simulink model "VF_Speed"  (R2023b)
settings: Solver=ode23  StartTime=0.0  StopTime=4  MaxStep=1e-6  RelTol=1e-4
InitFcn:
  | Pn = 4;
  | Ld = 5.25e-3;
  | Lq = 12e-3;
  | R = 0.958;
  | flux = 0.1827;
  | J = 0.003;
  | B = 0.008;
  | Vdc = 311;
  | fpwm = 10e3;
  | Ts = 1e-5;
model workspace: external: MATLAB File D:\Simulink\Study\PMSM建模第三章\VF_Params.m (data not in the file)
libraries: spsDCVoltageSourceLib x1, powerlib_extras x1, spsPermanentMagnetSynchronousMachineLib x1, simulink x1, spsUniversalBridgeLib x1, spspowerguiLib x1
settings Model: Creator=123  LastModifiedBy=123
settings ModelReferenceCC: EnableRefExpFcnMdlSchedulingChecks=on

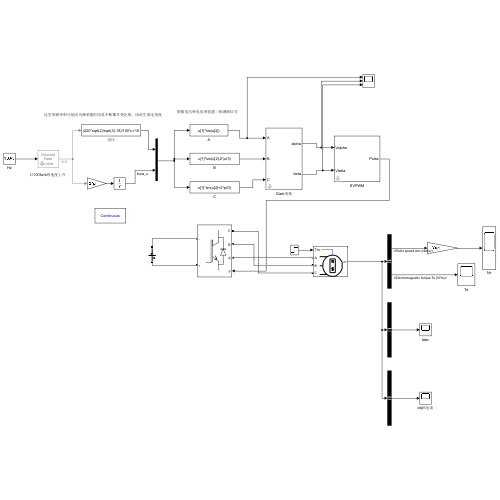
[thumbnail: Simulink's stored preview of the top-level diagram]
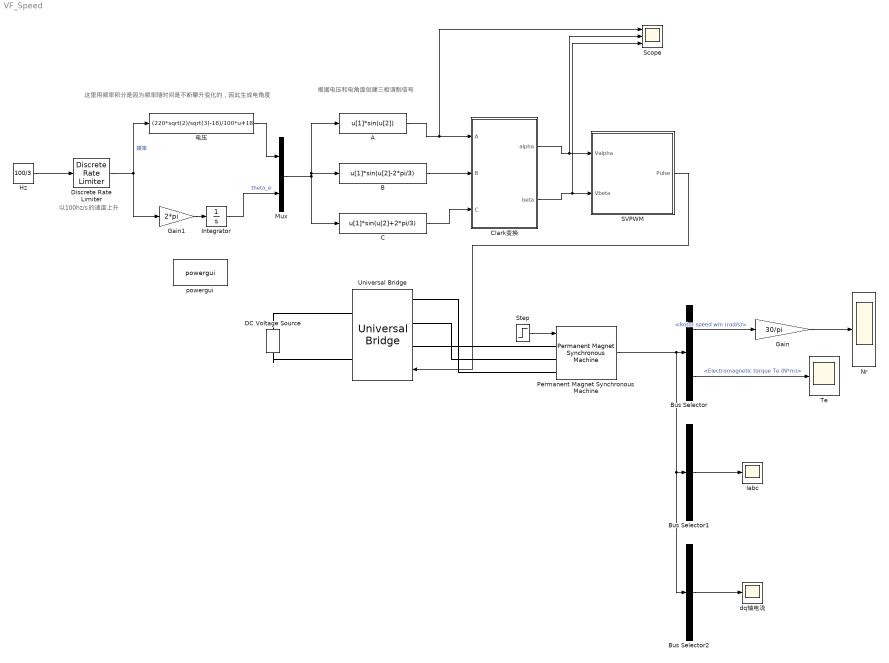
== system VF_Speed ==
  note: 以100hz/s的速度上升
  note: 这里用频率积分是因为频率随时间是不断攀升变化的，因此生成电角度
  note: 根据电压和电角度创建三相调制信号
  A : Fcn  Expr=u[1]*sin(u[2])
  B : Fcn  Expr=u[1]*sin(u[2]-2*pi/3)
  Bus Selector : BusSelector  OutputSignals=Rotor speed wm (rad/s),Electromagnetic torque Te (N*m)
  Bus Selector1 : BusSelector  OutputSignals=Stator current is_a (A),Stator current is_b (A),Stator current is_c (A)  OutputAsBus=on
  Bus Selector2 : BusSelector  OutputSignals=Stator current is_d (A),Stator current is_q (A)  OutputAsBus=on
  C : Fcn  Expr=u[1]*sin(u[2]+2*pi/3)
  Clark变换 : Subsystem
      mask DialogControl ParameterGroupVar Prompt: 参数
      mask Display:
      | port_label('input', 1, 'A');
      | port_label('input', 2, 'B');
      | port_label('input', 3, 'C');
      | port_label('output', 1, 'alpha');
      | port_label('output', 2, 'beta');
  DC Voltage Source : spsDCVoltageSourceLib/DC Voltage Source  Amplitude=Vdc  Measurements=None
  Discrete Rate Limiter : powerlib_extras/Discrete  Control Blocks/Discrete Rate Limiter  R=100  F=-100  Vinit=0  Ts=Ts
  Gain : Gain  Gain=30/pi
  Gain1 : Gain  Gain=2*pi
  Hz : Constant  Value=100/3
  Iabc : Scope
  Integrator : Integrator
  Mux : Mux  Inputs=2
  Nr : Scope
  Permanent Magnet Synchronous Machine : spsPermanentMagnetSynchronousMachineLib/Permanent Magnet Synchronous Machine  NbPhases=3  FluxDistribution=Sinusoidal  RotorType=Salient-pole  MechanicalLoad=Torque Tm  PresetModel=No  ShowDetailedParameters=on  MeasurementBus=off  Resistance=R  Inductance=8.5e-3  dqInductances=[Ld,Lq]  La=0.000395  MachineConstant=Flux linkage established by magnets (V.s)  Flux=flux  VoltageCst=132.5525  TorqueCst=1.0962  Flat=120  Mechanical=[J B Pn 0]  PolePairs=4  InitialConditions=[0,0, 0,0]  InitialConditions5ph=[0 0 0 0 0 0]  RefAngle=Aligned with phase A axis (original Park)  IterativeDiscreteModel=Trapezoidal non iterative  TsBlock=-1  TsPowergui=0
  SVPWM : Subsystem  mask(SVPWM){udc_ref=Vdc, tpwm_ref=1/fpwm}
      mask prompts: udc_ref "DC bus voltage (V)"; tpwm_ref "PWM period (s)"
      mask help: Amplitude-invariant alpha/beta voltage references in volts. Pulse order: A upper, A lower, B upper, B lower, C upper, C lower. Ideal complementary gates; no dead time.
      mask Display: port_label('input',1,'Valpha');port_label('input',2,'Vbeta');port_label('output',1,'Pulse');
  Scope : Scope  NumInputPorts=3
  Step : Step  Time=0.5  After=10  SampleTime=0
  Te : Scope
  Universal Bridge : spsUniversalBridgeLib/Universal Bridge  Arms=3  SnubberResistance=1e5  SnubberCapacitance=inf  Device=IGBT / Diodes  Ron=1e-3  Lon=0  ForwardVoltages="[  0  0  ]"  ForwardVoltage=0  GTOparameters=[ 10e-6 , 20e-6 ]  IGBTparameters=[ 1e-6 , 2e-6 ]  Measurements=None  Measurements_2=None  converterType=Rectifier
  dq轴电流 : Scope
  powergui : spspowerguiLib/powergui  Priority=1  SimulationMode=Continuous  SampleTime=5e-6  frequency=60  Iterations=50  frequencyindice=0  Pbase=100e6  ErrMax=1e-4  UnitsV=kV  UnitsW=MW  buscounter=0  FunctionMessages=off  echomessages=off  EnableUseOfTLC=off  CurrentSourceSwitches=off  DisableSnubberDevices=off  DisableRonSwitches=off  DisableVfSwitches=off  DisplayEquations=off  AutomaticDiscreteSolvers=off  SolverType=Tustin/Backward Euler (TBE)  Interpol=off  ExternalGateDelay=off  methode=off  Ts=100  x0status=blocks  SPID=on  SwTol=0  HookPort=off  NonlinearTolerance=1e-4  nMaxIteration=100  ContinueOnMaxIteration=off  RestoreLinks=warning  ResistiveCurrentMeasurement=off  Frange=[0:2:500]  Ylog=off  Xlog=on  ShowGrid=off  save=off  variable=ZData  structure=0  ZoomFFT=off  StartTime=0.0  cycles=1  DisplayStyle=1  fundamental=60  FreqAxis=off  MaxFrequency=1000  frequencyindicesteady=1  RmsSteady=1  display=off
  电压 : Fcn  Expr=(220*sqrt(2)/sqrt(3)-18)/100*u+18
  wires:
  Hz/1 -> Discrete Rate Limiter/1
  Discrete Rate Limiter/1 -> Gain1/1, 电压/1  "频率"
  Clark变换/1(alpha) -> Scope/2, SVPWM/1(Valpha)
  Clark变换/2(beta) -> Scope/3, SVPWM/2(Vbeta)
  SVPWM/1(Pulse) -> Universal Bridge/1
  Bus Selector/1 -> Gain/1  "<Rotor speed wm (rad/s)>"
  Bus Selector/2 -> Te/1  "<Electromagnetic torque Te (N*m)>"
  Gain/1 -> Nr/1
  Permanent Magnet Synchronous Machine/1 -> Bus Selector2/1, Bus Selector1/1, Bus Selector/1
  Bus Selector1/1 -> Iabc/1
  Step/1 -> Permanent Magnet Synchronous Machine/1
  Mux/1 -> B/1, A/1, C/1
  A/1 -> Scope/1, Clark变换/1(A)
  B/1 -> Clark变换/2(B)
  C/1 -> Clark变换/3(C)
  电压/1 -> Mux/1
  Gain1/1 -> Integrator/1
  Integrator/1 -> Mux/2  "theta_e"
  Bus Selector2/1 -> dq轴电流/1
  connections:
  DC Voltage Source/RConn1 -- Universal Bridge/RConn1
  DC Voltage Source/LConn1 -- Universal Bridge/RConn2
  Universal Bridge/LConn3 -- Permanent Magnet Synchronous Machine/LConn3
  Universal Bridge/LConn2 -- Permanent Magnet Synchronous Machine/LConn2
  Universal Bridge/LConn1 -- Permanent Magnet Synchronous Machine/LConn1

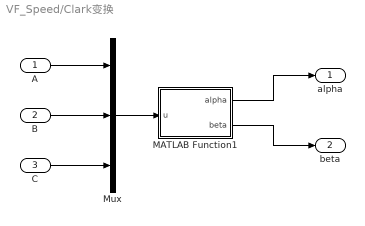
== system VF_Speed/Clark变换 ==
  A : Inport
  B : Inport  Port=2
  C : Inport  Port=3
  MATLAB Function1 : MATLAB Function  TreatAsAtomicUnit=on
  Mux : Mux  Inputs=3
  alpha : Outport
  beta : Outport  Port=2
  wires:
  A/1 -> Mux/1
  B/1 -> Mux/2
  C/1 -> Mux/3
  Mux/1 -> MATLAB Function1/1(u)
  MATLAB Function1/1(alpha) -> alpha/1
  MATLAB Function1/2(beta) -> beta/1

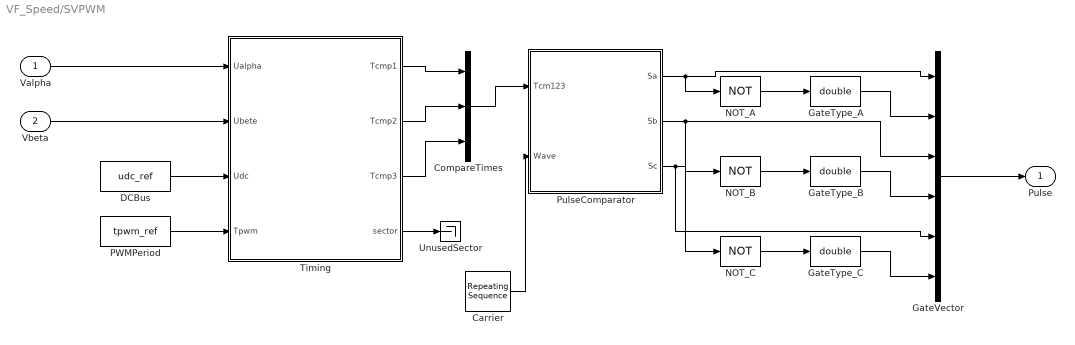
== system VF_Speed/SVPWM ==
  Valpha : Inport
  Vbeta : Inport  Port=2
  Carrier : simulink/Sources/Repeating Sequence  rep_seq_t=[0 tpwm_ref/2 tpwm_ref]  rep_seq_y=[0 tpwm_ref/2 0]
  CompareTimes : Mux  Inputs=3
  DCBus : Constant  Value=udc_ref
  GateType_A : DataTypeConversion  OutDataTypeStr=double  SaturateOnIntegerOverflow=off  RndMeth=Floor
  GateType_B : DataTypeConversion  OutDataTypeStr=double  SaturateOnIntegerOverflow=off  RndMeth=Floor
  GateType_C : DataTypeConversion  OutDataTypeStr=double  SaturateOnIntegerOverflow=off  RndMeth=Floor
  GateVector : Mux  Inputs=6
  NOT_A : Logic  Operator=NOT  AllPortsSameDT=off  OutDataTypeStr=boolean
  NOT_B : Logic  Operator=NOT  AllPortsSameDT=off  OutDataTypeStr=boolean
  NOT_C : Logic  Operator=NOT  AllPortsSameDT=off  OutDataTypeStr=boolean
  PWMPeriod : Constant  Value=tpwm_ref
  PulseComparator : Subsystem
  Timing : MATLAB Function  TreatAsAtomicUnit=on
  UnusedSector : Terminator
  Pulse : Outport
  wires:
  Valpha/1 -> Timing/1(Ualpha)
  Vbeta/1 -> Timing/2(Ubete)
  DCBus/1 -> Timing/3(Udc)
  PWMPeriod/1 -> Timing/4(Tpwm)
  Timing/1(Tcmp1) -> CompareTimes/1
  Timing/2(Tcmp2) -> CompareTimes/2
  Timing/3(Tcmp3) -> CompareTimes/3
  Timing/4(sector) -> UnusedSector/1
  CompareTimes/1 -> PulseComparator/1(Tcm123)
  Carrier/1 -> PulseComparator/2(Wave)
  PulseComparator/1(Sa) -> GateVector/1, NOT_A/1
  NOT_A/1 -> GateType_A/1
  GateType_A/1 -> GateVector/2
  PulseComparator/2(Sb) -> GateVector/3, NOT_B/1
  NOT_B/1 -> GateType_B/1
  GateType_B/1 -> GateVector/4
  PulseComparator/3(Sc) -> GateVector/5, NOT_C/1
  NOT_C/1 -> GateType_C/1
  GateType_C/1 -> GateVector/6
  GateVector/1 -> Pulse/1

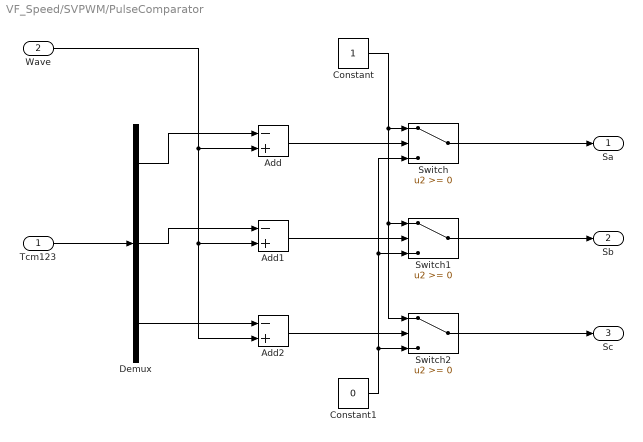
== system VF_Speed/SVPWM/PulseComparator ==
  Tcm123 : Inport
  Wave : Inport  Port=2
  Add : Sum  Inputs=-+
  Add1 : Sum  Inputs=-+
  Add2 : Sum  Inputs=-+
  Constant : Constant
  Constant1 : Constant  Value=0
  Demux : Demux  Outputs=3
  Switch : Switch  SaturateOnIntegerOverflow=off  InputSameDT=off
  Switch1 : Switch  SaturateOnIntegerOverflow=off  InputSameDT=off
  Switch2 : Switch  SaturateOnIntegerOverflow=off  InputSameDT=off
  Sa : Outport
  Sb : Outport  Port=2
  Sc : Outport  Port=3
  wires:
  Switch2/1 -> Sc/1
  Switch1/1 -> Sb/1
  Switch/1 -> Sa/1
  Constant1/1 -> Switch/3, Switch1/3, Switch2/3
  Constant/1 -> Switch/1, Switch1/1, Switch2/1
  Add/1 -> Switch/2
  Add1/1 -> Switch1/2
  Add2/1 -> Switch2/2
  Demux/3 -> Add2/1
  Demux/2 -> Add1/1
  Demux/1 -> Add/1
  Wave/1 -> Add2/2, Add1/2, Add/2
  Tcm123/1 -> Demux/1

== matlab function VF_Speed/Clark变换/MATLAB Function1 ==
  data: u input; alpha output; beta output
function [alpha, beta] = fcn(u)

alpha = (u(1)-0.5*(u(2)+u(3)))*2/3;
beta  = sqrt(3)/2*(u(2)-u(3))*2/3;

end

== matlab function VF_Speed/SVPWM/Timing ==
  data: Ualpha input; Tcmp1 output; Ubete input; Udc input; Tpwm input; Tcmp2 output; Tcmp3 output; sector output
function [Tcmp1,Tcmp2,Tcmp3,sector] = fcn(Ualpha,Ubete,Udc,Tpwm)

%变量初始化

Tcmp1 = 0;
Tcmp2 = 0;
Tcmp3 = 0;
sector = 0;
T1 = 0;
T2 = 0;

%扇区选择

Uref1 = Ubete;
Uref2 = (sqrt(3)*Ualpha - Ubete)/2;
Uref3 = (-sqrt(3)*Ualpha - Ubete)/2;

if(Uref1 > 0)
    sector = 1;
end
if(Uref2 > 0)
    sector = sector + 2;
end
if(Uref3 > 0)
    sector = sector + 4;
end

%非零矢量和零矢量作用时间

X = sqrt(3)*Ubete*Tpwm/Udc;
Y = Tpwm/Udc*(3/2*Ualpha + sqrt(3)/2*Ubete);
Z = Tpwm/Udc*(-3/2*Ualpha + sqrt(3)/2*Ubete);

switch(sector)
    case 1
        T1 = Z;T2 = Y;
    case 2
        T1 = Y;T2 = -X;
    case 3
        T1 = -Z;T2 = X;
    case 4
        T1 = -X;T2 = Z;
    case 5
        T1 = X;T2 = -Y;
    case 6
        T1 = -Y;T2 = -Z;
end

%过调制处理，变成占空比处理

if (T1+T2>Tpwm)
    scale = Tpwm/(T1+T2);
    T1 = T1*scale;
    T2 = T2*scale;
else
    T1 = T1;
    T2 = T2;
end

%扇区矢量切换点确定

ta = (Tpwm-(T1+T2))/4.0;
tb = ta+T1/2;
tc = tb+T2/2;

switch(sector)
    case 1
        Tcmp1 = tb;
        Tcmp2 = ta;
        Tcmp3 = tc;
    case 2
        Tcmp1 = ta;
        Tcmp2 = tc;
        Tcmp3 = tb;
    case 3
        Tcmp1 = ta;
        Tcmp2 = tb;
        Tcmp3 = tc;
    case 4
        Tcmp1 = tc;
        Tcmp2 = tb;
        Tcmp3 = ta;
    case 5
        Tcmp1 = tc;
        Tcmp2 = ta;
        Tcmp3 = tb;
    case 6
        Tcmp1 = tb;
        Tcmp2 = tc;
        Tcmp3 = ta;
end
end
